simulink library "Multibody_Parts_Lib"  (R2024a)
settings: Solver=VariableStepAuto  StartTime=0.0  StopTime=10.0  RelTol=1e-3
undefined symbols (not defined in the file or in its folder): b_gear_pd_asy, b_radius_asy, b_visc_frict_asy, bevel_angle_asy, bevel_angle_bf_asy, bevel_angle_fg_asy, f_gear_pd_asy, f_radius_asy, f_visc_frict_asy, g_radius_asy, g_visc_frict_asy, gear_ra_asy, gear_visc_frict_asy, Hand, Left, Local, pinion_pd_asy, screw_lead, worm_lead_angle_asy, worm_rad_asy, worm_visc_frict_asy, X, Y, Z
libraries: sm_lib x143, $bdroot x22, nesl_utility x16
(part 2 of 6)

== system Multibody_Parts_Lib/Gears ==
  Assemblies : Subsystem
  Bevel Gear : Subsystem  mask(Bevel Gear){gear_ra=0.125, gear_th=0.02, gear_ca=90/2, gear_hr=0.02, gear_rho=7000, gear_clr=[0.0 0.4 0.6], gear_opc=1, popup_markings=Two, mark_radius_range=[0.7 0.8], mark_angle_range=60, mark_color=[1 1 1]}
      mask prompts: gear_ra "Radius (m):"; gear_th "Thickness (m):"; gear_ca "Cone Angle (deg):"; gear_hr "Hole Radius (m):"; gear_rho "Density (kg/m^3):"; gear_clr "Color [RGB]:"; gear_opc "Opacity (0-1)"; popup_markings "Show Markings"; mark_radius_range "Radial Range [min max] (0-1)"; mark_angle_range "Sweep Angle [0-180] (deg)"; mark_color "Color [RGB]"
      mask help:
      | This block models a bevel gear with a hole for the shaft.
      |
      | The port C corresponds to the frame at the center of the gear.
      mask init:
      | gear_xsec = [gear_hr -gear_th/2;
      |              gear_ra -gear_th/2;
      |              gear_ra 0;
      |              gear_ra-gear_th/2/tand((90-gear_ca))  gear_th/2;
      |              gear_hr gear_th/2];
      | mark_xsec =  [
      |     gear_ra*max(mark_radius_range) gear_th/1.9; 
      |     gear_ra*min(mark_radius_range) gear_th/1.9; 
      |     gear_ra*min(mark_radius_range) -gear_th/1.9; 
      |     gear_ra*max(mark_radius_range) -gear_th/1.9];
      | 
      | mark_1_opc = 0;
      | mark_2_opc = 0;
      | 
      | if(popup_markings == 2)
      |     mark_1_opc = 1;
      | elseif(popup_markings == 3)
      |     mark_1_opc = 1;
      |     mark_2_opc = 1;
      | end
      mask TypeOptions popup_markings: None | One | Two
      mask Callback popup_markings:
      | maskObj = Simulink.Mask.get(gcb);
      | mkc_h = maskObj.getDialogControl('container_markings');
      | if strcmp(get_param(gcb,'popup_markings'),'None')
      |     mkc_h.Visible = 'off';
      | else
      |     mkc_h.Visible = 'on';
      | end
      | clear maskObj mkc_h
      mask Display: image('Bevel_Gear_IMAGE.png')
  Forces : Subsystem
  Gear : Subsystem  mask(Gear){popup_gear_type=External, gear_pd=0.125, gear_nt=12, gear_th=0.02, gear_rh=0.005, gear_rt=0.02, gear_rho=7000, gear_clr=[0.0 0.4 0.6], gear_opc=1, popup_ad_dd=Default, gear_ad=0.125/12, gear_dd=1.157*0.125/12, popup_markings=Two, mark_radius_range=[0.6 0.7], mark_angle_range=60, mark_color=[1 1 1]}
      mask prompts: popup_gear_type "Gear Type"; gear_pd "Pitch Diameter (m)"; gear_nt "Number of Teeth"; gear_th "Gear Thickness (m)"; gear_rh "Hole Radius (m)"; gear_rt "Outer Radius (m)"; gear_rho "Density (kg/m^3)"; gear_clr "Color [RGB]"; gear_opc "Opacity (0-1)"; popup_ad_dd "Addendum, Dedendum"; gear_ad "Addendum (m)"; gear_dd "Dedendum (m)"; popup_markings "Show Markings"; mark_radius_range "Radial Range [min max] (0-1)"; mark_angle_range "Sweep Angle [0-180] (deg)"; mark_color "Color [RGB]"
      mask help: This block models an external or internal involute tooth gear. The gear tooth profile assumes a pressure angle of 14.5 degrees.
      mask init:
      | if (strcmp(get_param(gcb,'popup_gear_type'),'External'))
      |     gear_holeORouter = gear_rh;
      | else
      |     gear_holeORouter = gear_rt;
      | end
      | 
      | if (strcmp(get_param(gcb,'popup_ad_dd'),'Default'))
      | gear_xsec = Extr_Data_Gear(...
      |     get_param(gcb,'popup_gear_type'),...
      |     gear_pd, gear_nt, gear_holeORouter);
      | else
      | gear_xsec = Extr_Data_Gear(...
      |     get_param(gcb,'popup_gear_type'),...
      |     gear_pd, gear_nt, gear_holeORouter, gear_ad, gear_dd);
      | end
      | 
      | mark_xsec =  [
      |     gear_pd/2*max(mark_radius_range) gear_th/1.9; 
      |     gear_pd/2*min(mark_radius_range) gear_th/1.9; 
      |     gear_pd/2*min(mark_radius_range) -gear_th/1.9; 
      |     gear_pd/2*max(mark_radius_range) -gear_th/1.9];
      | 
      | mark_1_opc = 0;
      | mark_2_opc = 0;
      | 
      | if(popup_markings == 2)
      |     mark_1_opc = 1;
      | elseif(popup_markings == 3)
      |     mark_1_opc = 1;
      |     mark_2_opc = 1;
      | end
      mask TypeOptions popup_gear_type: External | Internal
      mask Callback popup_gear_type:
      | maskObj = Simulink.Mask.get(gcb);
      | grh_h = maskObj.getParameter('gear_rh');
      | grt_h = maskObj.getParameter('gear_rt');
      | if strcmp(get_param(gcb,'popup_gear_type'),'External')
      |     grh_h.Visible = 'on';
      |     grt_h.Visible = 'off';
      | else
      |     grh_h.Visible = 'off';
      |     grt_h.Visible = 'on';
      | end
      | clear maskObj grh_h grt_h
      mask TypeOptions popup_ad_dd: Default | Specify
      mask Callback popup_ad_dd:
      | maskObj = Simulink.Mask.get(gcb);
      | gad_h = maskObj.getParameter('gear_ad');
      | gdd_h = maskObj.getParameter('gear_dd');
      | if strcmp(get_param(gcb,'popup_ad_dd'),'Default')
      |     gad_h.Visible = 'off';
      |     gdd_h.Visible = 'off';
      | else
      |     gad_h.Visible = 'on';
      |     gdd_h.Visible = 'on';
      | end
      | clear maskObj gad_h gdd_h
      mask TypeOptions popup_markings: None | One | Two
      mask Callback popup_markings:
      | maskObj = Simulink.Mask.get(gcb);
      | mkc_h = maskObj.getDialogControl('container_markings');
      | if strcmp(get_param(gcb,'popup_markings'),'None')
      |     mkc_h.Visible = 'off';
      | else
      |     mkc_h.Visible = 'on';
      | end
      | clear maskObj mkc_h
      mask DialogControl Control2 Prompt: Plot Profile
      mask DialogControl Control2 Callback:
      | v = get_param(gcb,'MaskWSVariables');
      | getMaskValue = containers.Map({v.Name}',{v.Value}');
      | 
      | if (strcmp(get_param(gcb,'popup_gear_type'),'External'))
      |     gear_holeORouter = getMaskValue('gear_rh');
      | else
      |     gear_holeORouter = getMaskValue('gear_rt');
      | end
      | 
      | if (strcmp(get_param(gcb,'popup_ad_dd'),'Default'))
      |     evalin('base',...
      |         sprintf('Extr_Data_Gear(''%s'',%s,%s,%s,''%s'');',...
      |         get_param(gcb,'popup_gear_type'),...
      |         num2str(getMaskValue('gear_pd')),...
      |         num2str(getMaskValue('gear_nt')),...
      |         num2str(gear_holeORouter),'plot'));
      | else
      |     evalin('base',...
      |         sprintf('Extr_Data_Gear(''%s'',%s,%s,%s,%s,%s,''%s'');',...
      |         get_param(gcb,'popup_gear_type'),...
      |         num2str(getMaskValue('gear_pd')),...
      |         num2str(getMaskValue('gear_nt')),...
      |         num2str(gear_holeORouter),...
      |         num2str(getMaskValue('gear_ad')),...
      |         num2str(getMaskValue('gear_dd')),'plot'));
      | end
      mask Display:
      | if(strcmpi(get_param(gcb,'popup_gear_type'),'Internal'))
      |     image('Gear_Internal_IMAGE.png');
      | else
      |     image('Gear_External_IMAGE.png');
      | end
  Rack : Subsystem  mask(Rack){rack_tp=0.052, rack_nt=15, rack_tb=0.02, rack_th=0.02, rack_rho=7000, rack_clr=[0.5 0.5 0.5], rack_opc=1, popup_ad_dd=Default, rack_ad=0.052/pi, rack_dd=1.157*0.052/pi}
      mask prompts: rack_tp "Teeth Pitch (m)"; rack_nt "Number of Teeth"; rack_tb "Thickness of Rack Base (m)"; rack_th "Thickness of Rack (m)"; rack_rho "Density (kg/m^3)"; rack_clr "Color [RGB]"; rack_opc "Opacity (0-1)"; popup_ad_dd "Addendum, Dedendum"; rack_ad "Addendum (m)"; rack_dd "Dedendum (m)"
      mask help: This block models a toothed bar (rack).
      mask init:
      | if (strcmp(get_param(gcb,'popup_ad_dd'),'Default'))
      | rack_xsec = Extr_Data_Rack(...
      |     rack_tp, rack_nt, rack_tb);
      | else
      | rack_xsec = Extr_Data_Rack(...
      |     rack_tp, rack_nt, rack_tb, rack_ad, rack_dd);
      | end
      mask TypeOptions popup_ad_dd: Default | Specify
      mask Callback popup_ad_dd:
      | maskObj = Simulink.Mask.get(gcb);
      | rad_h = maskObj.getParameter('rack_ad');
      | rdd_h = maskObj.getParameter('rack_dd');
      | if strcmp(get_param(gcb,'popup_ad_dd'),'Default')
      |     rad_h.Visible = 'off';
      |     rdd_h.Visible = 'off';
      | else
      |     rad_h.Visible = 'on';
      |     rdd_h.Visible = 'on';
      | end
      | clear maskObj rad_h rdd_h
      mask DialogControl Control2 Prompt: Plot Profile
      mask DialogControl Control2 Callback:
      | v = get_param(gcb,'MaskWSVariables');
      | getMaskValue = containers.Map({v.Name}',{v.Value}');
      | if (strcmp(get_param(gcb,'popup_ad_dd'),'Default'))
      |     evalin('base',...
      |         sprintf('Extr_Data_Rack(%s,%s,%s,''%s'');',...
      |         num2str(getMaskValue('rack_tp')),...
      |         num2str(getMaskValue('rack_nt')),...
      |         num2str(getMaskValue('rack_tb')),'plot'));
      | else
      |     evalin('base',...
      |         sprintf('Extr_Data_Rack(%s,%s,%s,%s,%s,''%s'');',...
      |         num2str(getMaskValue('rack_tp')),...
      |         num2str(getMaskValue('rack_nt')),...
      |         num2str(getMaskValue('rack_tb')),...
      |         num2str(getMaskValue('rack_ad')),...
      |         num2str(getMaskValue('rack_dd')),'plot'));
      | end
      mask Display: image('Rack_IMAGE.png')

== system Multibody_Parts_Lib/Linkages ==
  Cam Circles : Subsystem  mask(Cam from Two Circles){rad_b=0.02, rad_f=0.01, radhb=0.005, radhf=0.005, cam_len=0.05, cam_thickness=0.01, cam_rho=7000, cam_color=[0 0.4 0.6], cam_opc=1}
      mask prompts: cam_thickness "Thickness (m)"; cam_rho "Density (kg/m^3)"; cam_color "Color [RGB]"; cam_opc "Opacity (0-1)"
      mask help: Cam formed from two circles. Define radius of each circle, distance separating circle centers, and thickness of cam. The two interface frames are at the center of each circle. Frame F is along the +Z axis from frame B.
      mask init:
      | cam_xsec = Extr_Data_Cam_Circles(rad_b, rad_f, cam_len, radhb, radhf);
      mask DialogControl Control13 Prompt: Plot Profile
      mask DialogControl Control13 Callback:
      | v = get_param(gcb,'MaskWSVariables');
      | getMaskValue = containers.Map({v.Name}',{v.Value}');
      | evalin('base',...
      |     sprintf('Extr_Data_Cam_Circles(%s,%s,%s,%s,%s,''%s'');',...
      |     num2str(getMaskValue('rad_b')),...
      |     num2str(getMaskValue('rad_f')),...
      |     num2str(getMaskValue('cam_len')),...
      |     num2str(getMaskValue('radhb')),...
      |     num2str(getMaskValue('radhf')),'plot'));
      mask DialogControl Control3 Prompt: Circle B
      mask DialogControl Control4 Prompt: Circle F
      mask DialogControl Control5 Prompt: Radius (m)
      mask DialogControl text_radh Prompt: Hole Radius (m)
      mask DialogControl Control10 Prompt: Separation (m)
      mask Display: image('Cam_Circles_IMAGE.png')
  Link : Subsystem  mask(Link with Rounded Ends){link_len=0.1, link_width=0.025, link_radh=0.005, link_numh=2, link_thickness=0.01, link_rho=7000, link_color=[0 0.4 0.6], link_opc=1}
      mask prompts: link_len "Length (m)"; link_width "Width (m)"; link_radh "Hole Radius (m)"; link_numh "Number of Holes"; link_thickness "Thickness (m)"; link_rho "Density (kg/m^3)"; link_color "Color [RGB]"; link_opc "Opacity (0-1)"
      mask help: Link with rounded ends and arbitrary number of holes. Define outer dimensions, hole radius, and number of holes. The interface frames are at the center of the holes at either end of the link.
      mask init:
      | link_xsec = Extr_Data_LinkHoles(link_len, link_width, link_radh, link_numh);
      mask DialogControl Control12 Prompt: Plot Profile
      mask DialogControl Control12 Callback:
      | v = get_param(gcb,'MaskWSVariables');
      | getMaskValue = containers.Map({v.Name}',{v.Value}');
      | evalin('base',...
      |     sprintf('Extr_Data_LinkHoles(%s,%s,%s,%s,''%s'');',...
      |     num2str(getMaskValue('link_len')),...
      |     num2str(getMaskValue('link_width')),...
      |     num2str(getMaskValue('link_radh')),...
      |     num2str(getMaskValue('link_numh')),'plot'));
      mask Display: image('Link_IMAGE.png')
  Link End : Subsystem  mask(Link End){circ_radout=0.025/2, circ_radin=0.005, popup_holelr=+X, deg_1=-90, deg_2=90, circ_len=0.01, circ_rho=7000, circ_color=[0 0.4 0.6], circ_opc=1}
      mask prompts: circ_radout "Outer Radius (m)"; circ_radin "Hole Radius (m)"; popup_holelr "Hole Side"; deg_1 "Start Angle (deg)"; deg_2 "Finish Angle (deg)"; circ_len "Thickness (m)"; circ_rho "Density (kg/m^3)"; circ_color "Color [RGB]"; circ_opc "Opacity (0-1)"
      mask help: Round end of Link. Define outer radius, hole radius, and hole placement. Port is at the hole center.
      mask init:
      | if(strcmpi(get_param(gcb,'popup_holelr'),'+X'));
      |     set_param(gcb,'deg_1','-90','deg_2','90');
      | else
      |     set_param(gcb,'deg_1','90','deg_2','270');
      | end
      | circ_xsec = Extr_Data_Ring(circ_radout, circ_radin, deg_1, deg_2);
      mask TypeOptions popup_holelr: -X | +X
      mask DialogControl Control12 Prompt: Plot Profile
      mask DialogControl Control12 Callback:
      | v = get_param(gcb,'MaskWSVariables');
      | getMaskValue = containers.Map({v.Name}',{v.Value}');
      | 
      | if(strcmp(get_param(gcb,'popup_holelr'),'+X'))
      |     evalin('base',...
      |         sprintf('Extr_Data_Ring(%s,%s,%s,%s,''%s'');',...
      |         num2str(getMaskValue('circ_radout')),...
      |         num2str(getMaskValue('circ_radin')),...
      |         '-90',...
      |         '90','plot'));
      | else
      |     evalin('base',...
      |         sprintf('Extr_Data_Ring(%s,%s,%s,%s,''%s'');',...
      |         num2str(getMaskValue('circ_radout')),...
      |         num2str(getMaskValue('circ_radin')),...
      |         '90',...
      |         '270','plot'));
      | end
      mask Display:
      | if(strcmp(get_param(gcb,'popup_holelr'),'+X'))
      |     image('Link_End_px_IMAGE.png');
      | else
      |     image('Link_End_nx_IMAGE.png');
      | end
  Link Seg 1 Hole : Subsystem  mask(Link Segment with 1 Hole){link_len=0.05, link_width=0.025, link_radh=0.005, link_holelr=+X, link_thickness=0.01, link_rho=7000, link_color=[0 0.4 0.6], link_opc=1}
      mask prompts: link_len "Length (m)"; link_width "Width (m)"; link_radh "Hole Radius (m)"; link_holelr "Hole Side"; link_thickness "Thickness (m)"; link_rho "Density (kg/m^3)"; link_color "Color [RGB]"; link_opc "Opacity (0-1)"
      mask help: Link segment with one hole. Define outer dimensions, hole radius, and which end of the segment has the hole. The interface ports are at either end of the link segment.
      mask init:
      | link_xsec = Extr_Data_Link1Hole(link_len, link_width, link_radh, get_param(gcb,'link_holelr'));
      mask TypeOptions link_holelr: -X | +X
      mask DialogControl Control12 Prompt: Plot Profile
      mask DialogControl Control12 Callback:
      | v = get_param(gcb,'MaskWSVariables');
      | getMaskValue = containers.Map({v.Name}',{v.Value}');
      | evalin('base',...
      |     sprintf('Extr_Data_Link1Hole(%s,%s,%s,''%s'',''%s'');',...
      |     num2str(getMaskValue('link_len')),...
      |     num2str(getMaskValue('link_width')),...
      |     num2str(getMaskValue('link_radh')),...
      |     get_param(gcb,'link_holelr'),'plot'));
      mask Display:
      | if(strcmp(get_param(gcb,'link_holelr'),'+X'))
      |     image('Link_Seg_1_Hole_px_IMAGE.png');
      | else
      |     image('Link_Seg_1_Hole_nx_IMAGE.png');
      | end
  Link Seg 2 Hole : Subsystem  mask(Link Segment with 2 Holes){link_len=0.05, link_width=0.025, link_radh=0.005, link_thickness=0.01, link_rho=7000, link_color=[0 0.4 0.6], link_opc=1}
      mask prompts: link_len "Length (m)"; link_width "Width (m)"; link_radh "Hole Radius (m)"; link_thickness "Thickness (m)"; link_rho "Density (kg/m^3)"; link_color "Color [RGB]"; link_opc "Opacity (0-1)"
      mask help: Link segment with one hole. Define outer dimensions and hole radius. The interface ports are at either end of the link segment.
      mask init:
      | link_xsec = Extr_Data_Link2Hole(link_len, link_width, link_radh);
      mask DialogControl Control12 Prompt: Plot Profile
      mask DialogControl Control12 Callback:
      | v = get_param(gcb,'MaskWSVariables');
      | getMaskValue = containers.Map({v.Name}',{v.Value}');
      | evalin('base',...
      |     sprintf('Extr_Data_Link2Hole(%s,%s,%s,''%s'');',...
      |     num2str(getMaskValue('link_len')),...
      |     num2str(getMaskValue('link_width')),...
      |     num2str(getMaskValue('link_radh')),'plot'));
      mask Display: image('Link_Seg_2_Hole_IMAGE.png');
  Triangle Link : Subsystem  mask(Triangular Link with Rounded Corners){link_len=0.1, link_height=0.05, link_xlen=0.33, link_radh=0.005, link_rado=0.0125, link_thickness=0.01, link_rho=7000, link_color=[0 0.4 0.6], link_opc=1}
      mask prompts: link_len "Length (m)"; link_height "Height (m)"; link_xlen "Center Hole Position (0-1)"; link_radh "Hole Radius (m)"; link_rado "Link Outer Radius (m)"; link_thickness "Thickness (m)"; link_rho "Density (kg/m^3)"; link_color "Color [RGB]"; link_opc "Opacity (0-1)"
      mask help: Triangular link with rounded ends and 3 holes. Define outer dimensions, hole radius, and number of holes. The interface frames are at the center of each of the three holes.
      mask init:
      | link_xsec = Extr_Data_TriangleRounded_Holes(link_len, link_height, link_xlen, link_radh, link_rado);
      mask DialogControl Control12 Prompt: Plot Profile
      mask DialogControl Control12 Callback:
      | v = get_param(gcb,'MaskWSVariables');
      | getMaskValue = containers.Map({v.Name}',{v.Value}');
      | evalin('base',...
      |     sprintf('Extr_Data_TriangleRounded_Holes(%s,%s,%s,%s,%s,''%s'');',...
      |     num2str(getMaskValue('link_len')),...
      |     num2str(getMaskValue('link_height')),...
      |     num2str(getMaskValue('link_xlen')),...
      |     num2str(getMaskValue('link_radh')),...
      |     num2str(getMaskValue('link_rado')),'plot'));
      mask Display: image('Triangle_Link_IMAGE.png')

== system Multibody_Parts_Lib/Basic/Brick 2 Port ==
  Solid : sm_lib/Body Elements/Brick Solid  BrickDimensions=len_xyz  BrickDimensionsUnits=m  ExportEntireGeometry=off  InertiaType=CalculateFromGeometry  BasedOnType=Density  Density=brick_rho  DensityUnits=kg/m^3  Mass=1  MassUnits=kg  CenterOfMass=[0 0 0]  CenterOfMassUnits=m  MomentsOfInertia=[1 1 1]  MomentsOfInertiaUnits=kg*m^2  ProductsOfInertia=[1 1 1]  ProductsOfInertiaUnits=kg*m^2  GraphicType=FromGeometry  MarkerShape=Sphere  MarkerSize=10  GraphicVisPropType=SimpleVisualProperties  GraphicDiffuseColor=brick_clr  GraphicOpacity=brick_opc  GraphicSpecularColor=[0.5 0.5 0.5 1.0]  GraphicAmbientColor=[0.15 0.15 0.15 1.0]  GraphicEmissiveColor=[0.0 0.0 0.0 1.0]  GraphicShininess=75  DoExposeReferenceFrame=on  SerializedFrames=<Frames/>
  Transform 1 : sm_lib/Frames and Transforms/Rigid Transform  RotationMethod=None  FollAlignAxisA=+X  BaseAlignAxisA=+Y  FollAlignAxisB=+Y  BaseAlignAxisB=+Z  RotationStandardAxis=+Z  RotationAngle=0.0  RotationAngleUnits=deg  RotationArbitraryAxis=[0 0 1]  RotationSequenceAxes=FollowerAxes  RotationSequence=XYX  RotationSequenceAngles=[0 0 0]  RotationSequenceAnglesUnits=deg  RotationMatrix=[1 0 0; 0 1 0; 0 0 1]  Quaternion=[1 0 0 0]  TranslationMethod=Cartesian  TranslationCartesianOffset=port1_offset  TranslationCartesianOffsetUnits=m  TranslationStandardAxis=+Z  TranslationStandardOffset=0  TranslationStandardOffsetUnits=m  TranslationROffset=0  TranslationROffsetUnits=m  TranslationThetaOffset=0  TranslationThetaOffsetUnits=deg  TranslationZOffset=0  TranslationZOffsetUnits=m
  Transform 2 : sm_lib/Frames and Transforms/Rigid Transform  RotationMethod=None  FollAlignAxisA=+X  BaseAlignAxisA=+Y  FollAlignAxisB=+Y  BaseAlignAxisB=+Z  RotationStandardAxis=+Z  RotationAngle=0.0  RotationAngleUnits=deg  RotationArbitraryAxis=[0 0 1]  RotationSequenceAxes=FollowerAxes  RotationSequence=XYX  RotationSequenceAngles=[0 0 0]  RotationSequenceAnglesUnits=deg  RotationMatrix=[1 0 0; 0 1 0; 0 0 1]  Quaternion=[1 0 0 0]  TranslationMethod=Cartesian  TranslationCartesianOffset=port2_offset  TranslationCartesianOffsetUnits=m  TranslationStandardAxis=+Z  TranslationStandardOffset=0  TranslationStandardOffsetUnits=m  TranslationROffset=0  TranslationROffsetUnits=m  TranslationThetaOffset=0  TranslationThetaOffsetUnits=deg  TranslationZOffset=0  TranslationZOffsetUnits=m
  1X : PMIOPort  Side=Left
  X2 : PMIOPort  Port=2  Side=Right
  connections:
  Transform 1/RConn1 -- 1X/RConn1
  Solid/RConn1 -- Transform 1/LConn1 -- Transform 2/LConn1
  X2/RConn1 -- Transform 2/RConn1

== system Multibody_Parts_Lib/Basic/Brick 3 Port ==
  Solid : sm_lib/Body Elements/Brick Solid  BrickDimensions=len_xyz  BrickDimensionsUnits=m  ExportEntireGeometry=off  InertiaType=CalculateFromGeometry  BasedOnType=Density  Density=brick_rho  DensityUnits=kg/m^3  Mass=1  MassUnits=kg  CenterOfMass=[0 0 0]  CenterOfMassUnits=m  MomentsOfInertia=[1 1 1]  MomentsOfInertiaUnits=kg*m^2  ProductsOfInertia=[1 1 1]  ProductsOfInertiaUnits=kg*m^2  GraphicType=FromGeometry  MarkerShape=Sphere  MarkerSize=10  GraphicVisPropType=SimpleVisualProperties  GraphicDiffuseColor=brick_clr  GraphicOpacity=brick_opc  GraphicSpecularColor=[0.5 0.5 0.5 1.0]  GraphicAmbientColor=[0.15 0.15 0.15 1.0]  GraphicEmissiveColor=[0.0 0.0 0.0 1.0]  GraphicShininess=75  DoExposeReferenceFrame=on  SerializedFrames=<Frames/>
  Transform 1 : sm_lib/Frames and Transforms/Rigid Transform  RotationMethod=None  FollAlignAxisA=+X  BaseAlignAxisA=+Y  FollAlignAxisB=+Y  BaseAlignAxisB=+Z  RotationStandardAxis=+Z  RotationAngle=0.0  RotationAngleUnits=deg  RotationArbitraryAxis=[0 0 1]  RotationSequenceAxes=FollowerAxes  RotationSequence=XYX  RotationSequenceAngles=[0 0 0]  RotationSequenceAnglesUnits=deg  RotationMatrix=[1 0 0; 0 1 0; 0 0 1]  Quaternion=[1 0 0 0]  TranslationMethod=Cartesian  TranslationCartesianOffset=port1_offset  TranslationCartesianOffsetUnits=m  TranslationStandardAxis=+Z  TranslationStandardOffset=0  TranslationStandardOffsetUnits=m  TranslationROffset=0  TranslationROffsetUnits=m  TranslationThetaOffset=0  TranslationThetaOffsetUnits=deg  TranslationZOffset=0  TranslationZOffsetUnits=m
  Transform 2 : sm_lib/Frames and Transforms/Rigid Transform  RotationMethod=None  FollAlignAxisA=+X  BaseAlignAxisA=+Y  FollAlignAxisB=+Y  BaseAlignAxisB=+Z  RotationStandardAxis=+Z  RotationAngle=0.0  RotationAngleUnits=deg  RotationArbitraryAxis=[0 0 1]  RotationSequenceAxes=FollowerAxes  RotationSequence=XYX  RotationSequenceAngles=[0 0 0]  RotationSequenceAnglesUnits=deg  RotationMatrix=[1 0 0; 0 1 0; 0 0 1]  Quaternion=[1 0 0 0]  TranslationMethod=Cartesian  TranslationCartesianOffset=port2_offset  TranslationCartesianOffsetUnits=m  TranslationStandardAxis=+Z  TranslationStandardOffset=0  TranslationStandardOffsetUnits=m  TranslationROffset=0  TranslationROffsetUnits=m  TranslationThetaOffset=0  TranslationThetaOffsetUnits=deg  TranslationZOffset=0  TranslationZOffsetUnits=m
  Transform 3 : sm_lib/Frames and Transforms/Rigid Transform  RotationMethod=None  FollAlignAxisA=+X  BaseAlignAxisA=+Y  FollAlignAxisB=+Y  BaseAlignAxisB=+Z  RotationStandardAxis=+Z  RotationAngle=0.0  RotationAngleUnits=deg  RotationArbitraryAxis=[0 0 1]  RotationSequenceAxes=FollowerAxes  RotationSequence=XYX  RotationSequenceAngles=[0 0 0]  RotationSequenceAnglesUnits=deg  RotationMatrix=[1 0 0; 0 1 0; 0 0 1]  Quaternion=[1 0 0 0]  TranslationMethod=Cartesian  TranslationCartesianOffset=port3_offset  TranslationCartesianOffsetUnits=m  TranslationStandardAxis=+Z  TranslationStandardOffset=0  TranslationStandardOffsetUnits=m  TranslationROffset=0  TranslationROffsetUnits=m  TranslationThetaOffset=0  TranslationThetaOffsetUnits=deg  TranslationZOffset=0  TranslationZOffsetUnits=m
  1X : PMIOPort  Side=Left
  X2 : PMIOPort  Port=2  Side=Right
  X3 : PMIOPort  Port=3  Side=Right
  connections:
  X2/RConn1 -- Transform 2/RConn1
  Transform 1/LConn1 -- Transform 3/LConn1 -- Solid/RConn1 -- Transform 2/LConn1
  Transform 1/RConn1 -- 1X/RConn1
  X3/RConn1 -- Transform 3/RConn1

== system Multibody_Parts_Lib/Basic/Cone ==
  Cone : sm_lib/Body Elements/Revolved Solid  RevolutionCrossSection=frcon_xsec  RevolutionCrossSectionUnits=m  RevolutionExtent=Custom  RevolutionAngle=cone_angle_range(2)-cone_angle_range(1)  RevolutionAngleUnits=deg  ExportConvexHullGeometry=off  InertiaType=CalculateFromGeometry  BasedOnType=Density  Density=cone_rho  DensityUnits=kg/(m^3)  Mass=1  MassUnits=kg  CenterOfMass=[0 0 0]  CenterOfMassUnits=m  MomentsOfInertia=[1 1 1]  MomentsOfInertiaUnits=kg*m^2  ProductsOfInertia=[0 0 0]  ProductsOfInertiaUnits=kg*m^2  GraphicType=FromGeometry  MarkerShape=Sphere  MarkerSize=10  GraphicVisPropType=SimpleVisualProperties  GraphicDiffuseColor=cone_clr  GraphicOpacity=cone_opc  GraphicSpecularColor=[0.5 0.5 0.5 1.0]  GraphicAmbientColor=[0.15 0.15 0.15 1.0]  GraphicEmissiveColor=[0.0 0.0 0.0 1.0]  GraphicShininess=75  DoExposeReferenceFrame=on  SerializedFrames=<Frames/>
  Mark1 : sm_lib/Body Elements/Revolved Solid  RevolutionCrossSection=mark_xsec  RevolutionCrossSectionUnits=m  RevolutionExtent=Custom  RevolutionAngle=mark_angle_range  RevolutionAngleUnits=deg  ExportConvexHullGeometry=off  InertiaType=CalculateFromGeometry  BasedOnType=Density  Density=0  DensityUnits=kg/m^3  Mass=1  MassUnits=kg  CenterOfMass=[0 0 0]  CenterOfMassUnits=m  MomentsOfInertia=[1 1 1]  MomentsOfInertiaUnits=kg*m^2  ProductsOfInertia=[1 1 1]  ProductsOfInertiaUnits=kg*m^2  GraphicType=FromGeometry  MarkerShape=Sphere  MarkerSize=10  GraphicVisPropType=SimpleVisualProperties  GraphicDiffuseColor=mark_color  GraphicOpacity=mark_1_opc  GraphicSpecularColor=[0.5 0.5 0.5 1.0]  GraphicAmbientColor=[0.15 0.15 0.15 1.0]  GraphicEmissiveColor=[0.0 0.0 0.0 1.0]  GraphicShininess=75  DoExposeReferenceFrame=on  SerializedFrames=<Frames/>
  Mark2 : sm_lib/Body Elements/Revolved Solid  RevolutionCrossSection=mark_xsec  RevolutionCrossSectionUnits=m  RevolutionExtent=Custom  RevolutionAngle=mark_angle_range  RevolutionAngleUnits=deg  ExportConvexHullGeometry=off  InertiaType=CalculateFromGeometry  BasedOnType=Density  Density=0  DensityUnits=kg/m^3  Mass=1  MassUnits=kg  CenterOfMass=[0 0 0]  CenterOfMassUnits=m  MomentsOfInertia=[1 1 1]  MomentsOfInertiaUnits=kg*m^2  ProductsOfInertia=[1 1 1]  ProductsOfInertiaUnits=kg*m^2  GraphicType=FromGeometry  MarkerShape=Sphere  MarkerSize=10  GraphicVisPropType=SimpleVisualProperties  GraphicDiffuseColor=mark_color  GraphicOpacity=mark_2_opc  GraphicSpecularColor=[0.5 0.5 0.5 1.0]  GraphicAmbientColor=[0.15 0.15 0.15 1.0]  GraphicEmissiveColor=[0.0 0.0 0.0 1.0]  GraphicShininess=75  DoExposeReferenceFrame=on  SerializedFrames=<Frames/>
  Transform Mark 2 : sm_lib/Frames and Transforms/Rigid Transform  RotationMethod=StandardAxis  FollAlignAxisA=+X  BaseAlignAxisA=+Y  FollAlignAxisB=+Y  BaseAlignAxisB=+Z  RotationStandardAxis=+Z  RotationAngle=180  RotationAngleUnits=deg  RotationArbitraryAxis=[0 0 1]  RotationSequenceAxes=FollowerAxes  RotationSequence=XYX  RotationSequenceAngles=[0 0 0]  RotationSequenceAnglesUnits=deg  RotationMatrix=[1 0 0; 0 1 0; 0 0 1]  Quaternion=[1 0 0 0]  TranslationMethod=None  TranslationCartesianOffset=[0 0 0]  TranslationCartesianOffsetUnits=m  TranslationStandardAxis=+Z  TranslationStandardOffset=0  TranslationStandardOffsetUnits=m  TranslationROffset=0  TranslationROffsetUnits=m  TranslationThetaOffset=0  TranslationThetaOffsetUnits=deg  TranslationZOffset=0  TranslationZOffsetUnits=m
  Transform Sweep Angle : sm_lib/Frames and Transforms/Rigid Transform  RotationMethod=StandardAxis  FollAlignAxisA=+X  BaseAlignAxisA=+Y  FollAlignAxisB=+Y  BaseAlignAxisB=+Z  RotationStandardAxis=+Z  RotationAngle=(cone_angle_range(2)+cone_angle_range(1))/2  RotationAngleUnits=deg  RotationArbitraryAxis=[0 0 1]  RotationSequenceAxes=FollowerAxes  RotationSequence=XYX  RotationSequenceAngles=[0 0 0]  RotationSequenceAnglesUnits=deg  RotationMatrix=[1 0 0; 0 1 0; 0 0 1]  Quaternion=[1 0 0 0]  TranslationMethod=None  TranslationCartesianOffset=[0 0 0]  TranslationCartesianOffsetUnits=m  TranslationStandardAxis=+Z  TranslationStandardOffset=0  TranslationStandardOffsetUnits=m  TranslationROffset=0  TranslationROffsetUnits=m  TranslationThetaOffset=0  TranslationThetaOffsetUnits=deg  TranslationZOffset=0  TranslationZOffsetUnits=m
  C : PMIOPort  Side=Right
  connections:
  Transform Mark 2/LConn1 -- Transform Sweep Angle/LConn1 -- C/RConn1 -- Mark1/RConn1
  Transform Mark 2/RConn1 -- Mark2/RConn1
  Cone/RConn1 -- Transform Sweep Angle/RConn1

== system Multibody_Parts_Lib/Basic/Cylinder ==
  Cylinder : sm_lib/Body Elements/Revolved Solid  RevolutionCrossSection=cyl_xsec  RevolutionCrossSectionUnits=m  RevolutionExtent=Full  RevolutionAngle=355  RevolutionAngleUnits=deg  ExportConvexHullGeometry=off  InertiaType=CalculateFromGeometry  BasedOnType=Density  Density=cyl_rho  DensityUnits=kg/(m^3)  Mass=1  MassUnits=kg  CenterOfMass=[0 0 0]  CenterOfMassUnits=m  MomentsOfInertia=[1 1 1]  MomentsOfInertiaUnits=kg*m^2  ProductsOfInertia=[0 0 0]  ProductsOfInertiaUnits=kg*m^2  GraphicType=FromGeometry  MarkerShape=Sphere  MarkerSize=10  GraphicVisPropType=SimpleVisualProperties  GraphicDiffuseColor=cyl_clr  GraphicOpacity=cyl_opc  GraphicSpecularColor=[0.5 0.5 0.5 1.0]  GraphicAmbientColor=[0.15 0.15 0.15 1.0]  GraphicEmissiveColor=[0.0 0.0 0.0 1.0]  GraphicShininess=75  DoExposeReferenceFrame=on  SerializedFrames=<Frames/>
  Mark1 : sm_lib/Body Elements/Revolved Solid  RevolutionCrossSection=mark_xsec  RevolutionCrossSectionUnits=m  RevolutionExtent=Custom  RevolutionAngle=mark_angle_range  RevolutionAngleUnits=deg  ExportConvexHullGeometry=off  InertiaType=CalculateFromGeometry  BasedOnType=Density  Density=0  DensityUnits=kg/m^3  Mass=1  MassUnits=kg  CenterOfMass=[0 0 0]  CenterOfMassUnits=m  MomentsOfInertia=[1 1 1]  MomentsOfInertiaUnits=kg*m^2  ProductsOfInertia=[1 1 1]  ProductsOfInertiaUnits=kg*m^2  GraphicType=FromGeometry  MarkerShape=Sphere  MarkerSize=10  GraphicVisPropType=SimpleVisualProperties  GraphicDiffuseColor=mark_color  GraphicOpacity=mark_1_opc  GraphicSpecularColor=[0.5 0.5 0.5 1.0]  GraphicAmbientColor=[0.15 0.15 0.15 1.0]  GraphicEmissiveColor=[0.0 0.0 0.0 1.0]  GraphicShininess=75  DoExposeReferenceFrame=on  SerializedFrames=<Frames/>
  Mark2 : sm_lib/Body Elements/Revolved Solid  RevolutionCrossSection=mark_xsec  RevolutionCrossSectionUnits=m  RevolutionExtent=Custom  RevolutionAngle=mark_angle_range  RevolutionAngleUnits=deg  ExportConvexHullGeometry=off  InertiaType=CalculateFromGeometry  BasedOnType=Density  Density=0  DensityUnits=kg/m^3  Mass=1  MassUnits=kg  CenterOfMass=[0 0 0]  CenterOfMassUnits=m  MomentsOfInertia=[1 1 1]  MomentsOfInertiaUnits=kg*m^2  ProductsOfInertia=[1 1 1]  ProductsOfInertiaUnits=kg*m^2  GraphicType=FromGeometry  MarkerShape=Sphere  MarkerSize=10  GraphicVisPropType=SimpleVisualProperties  GraphicDiffuseColor=mark_color  GraphicOpacity=mark_2_opc  GraphicSpecularColor=[0.5 0.5 0.5 1.0]  GraphicAmbientColor=[0.15 0.15 0.15 1.0]  GraphicEmissiveColor=[0.0 0.0 0.0 1.0]  GraphicShininess=75  DoExposeReferenceFrame=on  SerializedFrames=<Frames/>
  Transform Mark 2 : sm_lib/Frames and Transforms/Rigid Transform  RotationMethod=StandardAxis  FollAlignAxisA=+X  BaseAlignAxisA=+Y  FollAlignAxisB=+Y  BaseAlignAxisB=+Z  RotationStandardAxis=+Z  RotationAngle=180  RotationAngleUnits=deg  RotationArbitraryAxis=[0 0 1]  RotationSequenceAxes=FollowerAxes  RotationSequence=XYX  RotationSequenceAngles=[0 0 0]  RotationSequenceAnglesUnits=deg  RotationMatrix=[1 0 0; 0 1 0; 0 0 1]  Quaternion=[1 0 0 0]  TranslationMethod=None  TranslationCartesianOffset=[0 0 0]  TranslationCartesianOffsetUnits=m  TranslationStandardAxis=+Z  TranslationStandardOffset=0  TranslationStandardOffsetUnits=m  TranslationROffset=0  TranslationROffsetUnits=m  TranslationThetaOffset=0  TranslationThetaOffsetUnits=deg  TranslationZOffset=0  TranslationZOffsetUnits=m
  C : PMIOPort  Side=Right
  connections:
  Transform Mark 2/RConn1 -- Mark2/RConn1
  Mark1/RConn1 -- C/RConn1 -- Transform Mark 2/LConn1 -- Cylinder/RConn1

== system Multibody_Parts_Lib/Basic/Mesh ==
  Solid : sm_lib/Body Elements/Extruded Solid  ExtrusionType=General  PolygonNumSides=3  PolygonOuterRadius=1  PolygonOuterRadiusUnits=m  ExportEntireGeometry=off  ExtrusionCrossSection=mesh_xsec  ExtrusionCrossSectionUnits=m  ExportConvexHullGeometry=off  ExtrusionLength=mesh_thickness  ExtrusionLengthUnits=m  InertiaType=CalculateFromGeometry  BasedOnType=Density  Density=mesh_rho  DensityUnits=kg/(m^3)  Mass=1  MassUnits=kg  CenterOfMass=[0 0 0]  CenterOfMassUnits=m  MomentsOfInertia=[1 1 1]  MomentsOfInertiaUnits=kg*m^2  ProductsOfInertia=[0 0 0]  ProductsOfInertiaUnits=kg*m^2  GraphicType=FromGeometry  MarkerShape=Sphere  MarkerSize=10  GraphicVisPropType=SimpleVisualProperties  GraphicDiffuseColor=mesh_color  GraphicOpacity=mesh_opc  GraphicSpecularColor=[0.5 0.5 0.5 1.0]  GraphicAmbientColor=[0.15 0.15 0.15 1.0]  GraphicEmissiveColor=[0.0 0.0 0.0 1.0]  GraphicShininess=75  DoExposeReferenceFrame=on  SerializedFrames=<Frames><Frame><Id>Frame1</Id><Value><Name>F</Name><Origin><Source>GeometricFeature</Source><FeatureName>top surface</FeatureName></Origin><PrimaryAxis><DefinedDirection>+Z</DefinedDirection><Source>ReferenceFrame</Source><SourceDirection>+Z</SourceDirection><FeatureName></FeatureName></PrimaryAxis><SecondaryAxis><DefinedDirection>+X</DefinedDirection><Source>ReferenceFrame</Source><SourceDirection>+X</SourceDirection><FeatureName></FeatureName></SecondaryAxis></Value></Frame><Frame><Id>Frame2</Id><Value><Name>B</Name><Origin><Source>GeometricFeature</Source><FeatureName>bottom surface</FeatureName></Origin><PrimaryAxis><DefinedDirection>+Z</DefinedDirection><Source>ReferenceFrame</Source><SourceDirection>+Z</SourceDirection><FeatureName></FeatureName></PrimaryAxis><SecondaryAxis><DefinedDirection>+X</DefinedDirection><Source>ReferenceFrame</Source><SourceDirection>+X</SourceDirection><FeatureName></FeatureName></SecondaryAxis></Value></Frame></Frames>
  F : PMIOPort  Side=Right
  R : PMIOPort  Port=2  Side=Left
  B : PMIOPort  Port=3  Side=Right
  connections:
  Solid/RConn1 -- R/RConn1
  F/RConn1 -- Solid/LConn1
  B/RConn1 -- Solid/LConn2

== system Multibody_Parts_Lib/Basic/Pulley ==
  Mark1 : sm_lib/Body Elements/Revolved Solid  RevolutionCrossSection=mark_xsec  RevolutionCrossSectionUnits=m  RevolutionExtent=Custom  RevolutionAngle=mark_angle_range  RevolutionAngleUnits=deg  ExportConvexHullGeometry=off  InertiaType=CalculateFromGeometry  BasedOnType=Density  Density=0  DensityUnits=kg/m^3  Mass=1  MassUnits=kg  CenterOfMass=[0 0 0]  CenterOfMassUnits=m  MomentsOfInertia=[1 1 1]  MomentsOfInertiaUnits=kg*m^2  ProductsOfInertia=[1 1 1]  ProductsOfInertiaUnits=kg*m^2  GraphicType=FromGeometry  MarkerShape=Sphere  MarkerSize=10  GraphicVisPropType=SimpleVisualProperties  GraphicDiffuseColor=mark_color  GraphicOpacity=mark_1_opc  GraphicSpecularColor=[0.5 0.5 0.5 1.0]  GraphicAmbientColor=[0.15 0.15 0.15 1.0]  GraphicEmissiveColor=[0.0 0.0 0.0 1.0]  GraphicShininess=75  DoExposeReferenceFrame=on  SerializedFrames=<Frames/>
  Mark2 : sm_lib/Body Elements/Revolved Solid  RevolutionCrossSection=mark_xsec  RevolutionCrossSectionUnits=m  RevolutionExtent=Custom  RevolutionAngle=mark_angle_range  RevolutionAngleUnits=deg  ExportConvexHullGeometry=off  InertiaType=CalculateFromGeometry  BasedOnType=Density  Density=0  DensityUnits=kg/m^3  Mass=1  MassUnits=kg  CenterOfMass=[0 0 0]  CenterOfMassUnits=m  MomentsOfInertia=[1 1 1]  MomentsOfInertiaUnits=kg*m^2  ProductsOfInertia=[1 1 1]  ProductsOfInertiaUnits=kg*m^2  GraphicType=FromGeometry  MarkerShape=Sphere  MarkerSize=10  GraphicVisPropType=SimpleVisualProperties  GraphicDiffuseColor=mark_color  GraphicOpacity=mark_2_opc  GraphicSpecularColor=[0.5 0.5 0.5 1.0]  GraphicAmbientColor=[0.15 0.15 0.15 1.0]  GraphicEmissiveColor=[0.0 0.0 0.0 1.0]  GraphicShininess=75  DoExposeReferenceFrame=on  SerializedFrames=<Frames/>
  Pulley : sm_lib/Body Elements/Revolved Solid  RevolutionCrossSection=pulley_xsec  RevolutionCrossSectionUnits=m  RevolutionExtent=Full  RevolutionAngle=355  RevolutionAngleUnits=deg  ExportConvexHullGeometry=off  InertiaType=CalculateFromGeometry  BasedOnType=Density  Density=pulley_rho  DensityUnits=kg/(m^3)  Mass=1  MassUnits=kg  CenterOfMass=[0 0 0]  CenterOfMassUnits=m  MomentsOfInertia=[1 1 1]  MomentsOfInertiaUnits=kg*m^2  ProductsOfInertia=[0 0 0]  ProductsOfInertiaUnits=kg*m^2  GraphicType=FromGeometry  MarkerShape=Sphere  MarkerSize=10  GraphicVisPropType=SimpleVisualProperties  GraphicDiffuseColor=pulley_clr  GraphicOpacity=pulley_opc  GraphicSpecularColor=[0.5 0.5 0.5 1.0]  GraphicAmbientColor=[0.15 0.15 0.15 1.0]  GraphicEmissiveColor=[0.0 0.0 0.0 1.0]  GraphicShininess=75  DoExposeReferenceFrame=on  SerializedFrames=<Frames/>
  Transform Mark 2 : sm_lib/Frames and Transforms/Rigid Transform  RotationMethod=StandardAxis  FollAlignAxisA=+X  BaseAlignAxisA=+Y  FollAlignAxisB=+Y  BaseAlignAxisB=+Z  RotationStandardAxis=+Z  RotationAngle=180  RotationAngleUnits=deg  RotationArbitraryAxis=[0 0 1]  RotationSequenceAxes=FollowerAxes  RotationSequence=XYX  RotationSequenceAngles=[0 0 0]  RotationSequenceAnglesUnits=deg  RotationMatrix=[1 0 0; 0 1 0; 0 0 1]  Quaternion=[1 0 0 0]  TranslationMethod=None  TranslationCartesianOffset=[0 0 0]  TranslationCartesianOffsetUnits=m  TranslationStandardAxis=+Z  TranslationStandardOffset=0  TranslationStandardOffsetUnits=m  TranslationROffset=0  TranslationROffsetUnits=m  TranslationThetaOffset=0  TranslationThetaOffsetUnits=deg  TranslationZOffset=0  TranslationZOffsetUnits=m
  Transform Swap Z : sm_lib/Frames and Transforms/Rigid Transform  RotationMethod=None  FollAlignAxisA=+X  BaseAlignAxisA=+Y  FollAlignAxisB=+Y  BaseAlignAxisB=+Z  RotationStandardAxis=+X  RotationAngle=180  RotationAngleUnits=deg  RotationArbitraryAxis=[0 0 1]  RotationSequenceAxes=FollowerAxes  RotationSequence=XYX  RotationSequenceAngles=[0 0 0]  RotationSequenceAnglesUnits=deg  RotationMatrix=[1 0 0; 0 1 0; 0 0 1]  Quaternion=[1 0 0 0]  TranslationMethod=None  TranslationCartesianOffset=[0 0 0]  TranslationCartesianOffsetUnits=m  TranslationStandardAxis=+Z  TranslationStandardOffset=0  TranslationStandardOffsetUnits=m  TranslationROffset=0  TranslationROffsetUnits=m  TranslationThetaOffset=0  TranslationThetaOffsetUnits=deg  TranslationZOffset=0  TranslationZOffsetUnits=m
  C : PMIOPort  Side=Right
  R : PMIOPort  Port=2  Side=Left
  connections:
  Pulley/RConn1 -- Transform Mark 2/LConn1 -- Transform Swap Z/LConn1 -- C/RConn1 -- Mark1/RConn1
  Transform Mark 2/RConn1 -- Mark2/RConn1
  R/RConn1 -- Transform Swap Z/RConn1

== system Multibody_Parts_Lib/Basic/Rod ==
  Mark1 : sm_lib/Body Elements/Revolved Solid  RevolutionCrossSection=mark_xsec  RevolutionCrossSectionUnits=m  RevolutionExtent=Custom  RevolutionAngle=mark_angle_range  RevolutionAngleUnits=deg  ExportConvexHullGeometry=off  InertiaType=CalculateFromGeometry  BasedOnType=Density  Density=0  DensityUnits=kg/m^3  Mass=1  MassUnits=kg  CenterOfMass=[0 0 0]  CenterOfMassUnits=m  MomentsOfInertia=[1 1 1]  MomentsOfInertiaUnits=kg*m^2  ProductsOfInertia=[1 1 1]  ProductsOfInertiaUnits=kg*m^2  GraphicType=FromGeometry  MarkerShape=Sphere  MarkerSize=10  GraphicVisPropType=SimpleVisualProperties  GraphicDiffuseColor=mark_color  GraphicOpacity=mark_1_opc  GraphicSpecularColor=[0.5 0.5 0.5 1.0]  GraphicAmbientColor=[0.15 0.15 0.15 1.0]  GraphicEmissiveColor=[0.0 0.0 0.0 1.0]  GraphicShininess=75  DoExposeReferenceFrame=on  SerializedFrames=<Frames/>
  Mark2 : sm_lib/Body Elements/Revolved Solid  RevolutionCrossSection=mark_xsec  RevolutionCrossSectionUnits=m  RevolutionExtent=Custom  RevolutionAngle=mark_angle_range  RevolutionAngleUnits=deg  ExportConvexHullGeometry=off  InertiaType=CalculateFromGeometry  BasedOnType=Density  Density=0  DensityUnits=kg/m^3  Mass=1  MassUnits=kg  CenterOfMass=[0 0 0]  CenterOfMassUnits=m  MomentsOfInertia=[1 1 1]  MomentsOfInertiaUnits=kg*m^2  ProductsOfInertia=[1 1 1]  ProductsOfInertiaUnits=kg*m^2  GraphicType=FromGeometry  MarkerShape=Sphere  MarkerSize=10  GraphicVisPropType=SimpleVisualProperties  GraphicDiffuseColor=mark_color  GraphicOpacity=mark_2_opc  GraphicSpecularColor=[0.5 0.5 0.5 1.0]  GraphicAmbientColor=[0.15 0.15 0.15 1.0]  GraphicEmissiveColor=[0.0 0.0 0.0 1.0]  GraphicShininess=75  DoExposeReferenceFrame=on  SerializedFrames=<Frames/>
  Rod : sm_lib/Body Elements/Cylindrical Solid  CylinderRadius=rod_rad  CylinderRadiusUnits=m  CylinderLength=rod_len  CylinderLengthUnits=m  ExportEntireGeometry=off  InertiaType=CalculateFromGeometry  BasedOnType=Density  Density=rod_rho  DensityUnits=kg/(m^3)  Mass=1  MassUnits=kg  CenterOfMass=[0 0 0]  CenterOfMassUnits=m  MomentsOfInertia=[1 1 1]  MomentsOfInertiaUnits=kg*m^2  ProductsOfInertia=[0 0 0]  ProductsOfInertiaUnits=kg*m^2  GraphicType=FromGeometry  MarkerShape=Sphere  MarkerSize=10  GraphicVisPropType=SimpleVisualProperties  GraphicDiffuseColor=rod_color  GraphicOpacity=rod_opc  GraphicSpecularColor=[0.5 0.5 0.5 1.0]  GraphicAmbientColor=[0.15 0.15 0.15 1.0]  GraphicEmissiveColor=[0.0 0.0 0.0 1.0]  GraphicShininess=75  DoExposeReferenceFrame=on  SerializedFrames=<Frames/>
  Transform Mark 2 : sm_lib/Frames and Transforms/Rigid Transform  RotationMethod=StandardAxis  FollAlignAxisA=+X  BaseAlignAxisA=+Y  FollAlignAxisB=+Y  BaseAlignAxisB=+Z  RotationStandardAxis=+Z  RotationAngle=180  RotationAngleUnits=deg  RotationArbitraryAxis=[0 0 1]  RotationSequenceAxes=FollowerAxes  RotationSequence=XYX  RotationSequenceAngles=[0 0 0]  RotationSequenceAnglesUnits=deg  RotationMatrix=[1 0 0; 0 1 0; 0 0 1]  Quaternion=[1 0 0 0]  TranslationMethod=None  TranslationCartesianOffset=[0 0 0]  TranslationCartesianOffsetUnits=m  TranslationStandardAxis=+Z  TranslationStandardOffset=0  TranslationStandardOffsetUnits=m  TranslationROffset=0  TranslationROffsetUnits=m  TranslationThetaOffset=0  TranslationThetaOffsetUnits=deg  TranslationZOffset=0  TranslationZOffsetUnits=m
  Transform B : sm_lib/Frames and Transforms/Rigid Transform  RotationMethod=None  FollAlignAxisA=+X  BaseAlignAxisA=+Y  FollAlignAxisB=+Y  BaseAlignAxisB=+Z  RotationStandardAxis=+Z  RotationAngle=0.0  RotationAngleUnits=deg  RotationArbitraryAxis=[0 0 1]  RotationSequenceAxes=FollowerAxes  RotationSequence=XYX  RotationSequenceAngles=[0 0 0]  RotationSequenceAnglesUnits=deg  RotationMatrix=[1 0 0; 0 1 0; 0 0 1]  Quaternion=[1 0 0 0]  TranslationMethod=StandardAxis  TranslationCartesianOffset=[0 0 0]  TranslationCartesianOffsetUnits=m  TranslationStandardAxis=+Z  TranslationStandardOffset=rod_len/2*z_ori  TranslationStandardOffsetUnits=m  TranslationROffset=0  TranslationROffsetUnits=m  TranslationThetaOffset=0  TranslationThetaOffsetUnits=deg  TranslationZOffset=0  TranslationZOffsetUnits=m
  Transform F : sm_lib/Frames and Transforms/Rigid Transform  RotationMethod=None  FollAlignAxisA=+X  BaseAlignAxisA=+Y  FollAlignAxisB=+Y  BaseAlignAxisB=+Z  RotationStandardAxis=+Z  RotationAngle=0.0  RotationAngleUnits=deg  RotationArbitraryAxis=[0 0 1]  RotationSequenceAxes=FollowerAxes  RotationSequence=XYX  RotationSequenceAngles=[0 0 0]  RotationSequenceAnglesUnits=deg  RotationMatrix=[1 0 0; 0 1 0; 0 0 1]  Quaternion=[1 0 0 0]  TranslationMethod=StandardAxis  TranslationCartesianOffset=[0 0 0]  TranslationCartesianOffsetUnits=m  TranslationStandardAxis=+Z  TranslationStandardOffset=rod_len/2*z_ori  TranslationStandardOffsetUnits=m  TranslationROffset=0  TranslationROffsetUnits=m  TranslationThetaOffset=0  TranslationThetaOffsetUnits=deg  TranslationZOffset=0  TranslationZOffsetUnits=m
  B : PMIOPort  Side=Left
  F : PMIOPort  Port=2  Side=Right
  connections:
  Rod/RConn1 -- Transform B/RConn1 -- Transform F/LConn1 -- Mark1/RConn1 -- Transform Mark 2/LConn1
  Transform Mark 2/RConn1 -- Mark2/RConn1
  B/RConn1 -- Transform B/LConn1
  Transform F/RConn1 -- F/RConn1

== system Multibody_Parts_Lib/Basic/Sphere ==
  Arcs : Subsystem
  Rings : Subsystem
  Sphere : sm_lib/Body Elements/Spherical Solid  SphereRadius=sph_radius  SphereRadiusUnits=m  ExportEntireGeometry=off  InertiaType=CalculateFromGeometry  BasedOnType=Density  Density=sph_density  DensityUnits=kg/(m^3)  Mass=30e-3  MassUnits=kg  CenterOfMass=[0 0 0]  CenterOfMassUnits=m  MomentsOfInertia=[1 1 1]*1.358e-6  MomentsOfInertiaUnits=kg*m^2  ProductsOfInertia=[0 0 0]  ProductsOfInertiaUnits=kg*m^2  GraphicType=FromGeometry  MarkerShape=Sphere  MarkerSize=10  GraphicVisPropType=SimpleVisualProperties  GraphicDiffuseColor=[0.0 0.5 0.7]  GraphicOpacity=sph_opacity  GraphicSpecularColor=[0.5 0.5 0.5 1.0]  GraphicAmbientColor=[0.15 0.15 0.15 1.0]  GraphicEmissiveColor=[0.0 0.0 0.0 1.0]  GraphicShininess=75  DoExposeReferenceFrame=on  SerializedFrames=<Frames/>
  R : PMIOPort  Side=Left
  connections:
  Sphere/RConn1 -- Arcs/LConn1 -- Rings/LConn1 -- R/RConn1

== system Multibody_Parts_Lib/Extrusions/Box Fillet Tube ==
  Solid : sm_lib/Body Elements/Extruded Solid  ExtrusionType=General  PolygonNumSides=3  PolygonOuterRadius=1  PolygonOuterRadiusUnits=m  ExportEntireGeometry=off  ExtrusionCrossSection=box_xsec  ExtrusionCrossSectionUnits=m  ExportConvexHullGeometry=off  ExtrusionLength=box_len  ExtrusionLengthUnits=m  InertiaType=CalculateFromGeometry  BasedOnType=Density  Density=box_rho  DensityUnits=kg/(m^3)  Mass=1  MassUnits=kg  CenterOfMass=[0 0 0]  CenterOfMassUnits=m  MomentsOfInertia=[1 1 1]  MomentsOfInertiaUnits=kg*m^2  ProductsOfInertia=[0 0 0]  ProductsOfInertiaUnits=kg*m^2  GraphicType=FromGeometry  MarkerShape=Sphere  MarkerSize=10  GraphicVisPropType=SimpleVisualProperties  GraphicDiffuseColor=box_color  GraphicOpacity=box_opc  GraphicSpecularColor=[0.5 0.5 0.5 1.0]  GraphicAmbientColor=[0.15 0.15 0.15 1.0]  GraphicEmissiveColor=[0.0 0.0 0.0 1.0]  GraphicShininess=75  DoExposeReferenceFrame=on  SerializedFrames=<Frames/>
  Transform B : sm_lib/Frames and Transforms/Rigid Transform  RotationMethod=StandardAxis  FollAlignAxisA=+X  BaseAlignAxisA=+Y  FollAlignAxisB=+Y  BaseAlignAxisB=+Z  RotationStandardAxis=+Y  RotationAngle=90  RotationAngleUnits=deg  RotationArbitraryAxis=[0 0 1]  RotationSequenceAxes=FollowerAxes  RotationSequence=XYX  RotationSequenceAngles=[0 0 0]  RotationSequenceAnglesUnits=deg  RotationMatrix=[1 0 0; 0 1 0; 0 0 1]  Quaternion=[1 0 0 0]  TranslationMethod=StandardAxis  TranslationCartesianOffset=[0 0 0]  TranslationCartesianOffsetUnits=m  TranslationStandardAxis=+X  TranslationStandardOffset=box_len/2  TranslationStandardOffsetUnits=m  TranslationROffset=0  TranslationROffsetUnits=m  TranslationThetaOffset=0  TranslationThetaOffsetUnits=deg  TranslationZOffset=0  TranslationZOffsetUnits=m
  Transform F : sm_lib/Frames and Transforms/Rigid Transform  RotationMethod=StandardAxis  FollAlignAxisA=+X  BaseAlignAxisA=+Y  FollAlignAxisB=+Y  BaseAlignAxisB=+Z  RotationStandardAxis=+Y  RotationAngle=-90  RotationAngleUnits=deg  RotationArbitraryAxis=[0 0 1]  RotationSequenceAxes=FollowerAxes  RotationSequence=XYX  RotationSequenceAngles=[0 0 0]  RotationSequenceAnglesUnits=deg  RotationMatrix=[1 0 0; 0 1 0; 0 0 1]  Quaternion=[1 0 0 0]  TranslationMethod=StandardAxis  TranslationCartesianOffset=[0 0 0]  TranslationCartesianOffsetUnits=m  TranslationStandardAxis=+Z  TranslationStandardOffset=box_len/2  TranslationStandardOffsetUnits=m  TranslationROffset=0  TranslationROffsetUnits=m  TranslationThetaOffset=0  TranslationThetaOffsetUnits=deg  TranslationZOffset=0  TranslationZOffsetUnits=m
  F : PMIOPort  Side=Right
  B : PMIOPort  Port=2  Side=Left
  connections:
  B/RConn1 -- Transform B/LConn1
  Transform F/RConn1 -- F/RConn1
  Transform B/RConn1 -- Solid/RConn1 -- Transform F/LConn1
